simulink model "day11p2"  (R2026a)
(part 3 of 4)

  Subsystem7/1(cacheNew) -> Delay5/1
  Subsystem5/1(queue) -> Subsystem6/5(queue)
  Selector1/1 -> Subsystem6/4(rowStrings), Width1/1
  Width1/1 -> Gain1/1
  Constant1/1 -> Subsystem4/1(In1), Subsystem6/2(data), Selector1/1
  Delay3/1 -> Subsystem4/2(In2), Subsystem5/1(In1)
  Delay4/1 -> Subsystem4/3(In3), Subsystem5/2(In2)
  Subsystem6/2(cnt) -> Subsystem7/5(cnt), Accumulator1/1
  Gain1/1 -> Subsystem7/3(rowLen), Subsystem6/3(N)
  Subsystem5/2(queueLen) -> Subsystem6/6(queueLen)
  Accumulator1/1 -> Display1/1
  Subsystem6/1(cachedCnt) -> Subsystem7/4(cachedCnt)
  Subsystem6/4(queueLenNew) -> Delay4/1
  Accumulator2/1 -> Display2/1
  Subsystem9/2(queueLen) -> Subsystem10/6(queueLen)
  Constant2/1 -> Subsystem8/1(In1), Subsystem10/2(data), Selector2/1
  Selector2/1 -> Subsystem10/4(rowStrings), Width2/1
  Subsystem9/1(queue) -> Subsystem10/5(queue)
  Subsystem10/1(cachedCnt) -> Subsystem11/4(cachedCnt)
  Subsystem11/1(cacheNew) -> Delay8/1
  Subsystem10/4(queueLenNew) -> Delay7/1
  Subsystem10/3(queueNew) -> Delay6/1
  Delay7/1 -> Subsystem9/2(In2), Subsystem8/3(In3)
  Delay6/1 -> Subsystem9/1(In1), Subsystem8/2(In2)
  Width2/1 -> Gain2/1
  Delay8/1 -> Subsystem10/1(cache), Subsystem11/1(cache)
  Subsystem8/1(nodeIdx) -> Subsystem11/2(nodeIdx), Selector2/2
  Gain2/1 -> Subsystem11/3(rowLen), Subsystem10/3(N)
  Subsystem10/2(cnt) -> Subsystem11/5(cnt), Accumulator2/1
